simulink model "sf_aircraft"  (R2025b)
settings: configuration reference "SharedConfig" (kept outside this file)
PreLoadFcn:
  | load_system('sf_aircraft_lib.slx');
  | load_system('sf_aircraft_controller.slx');
model workspace (MAT data in the model file):
  reset_cmd = 0
values from neighbouring files (symbols this model uses):
  ActuatorModeType : value not decoded    [sf_aircraft_dd.sldd]
undefined symbols (not defined in the file or in its folder): Left, noise_factor, Right
libraries: simulink x15, sf_aircraft_lib x4, SignalEditorBlockLib x1
(part 2 of 2)

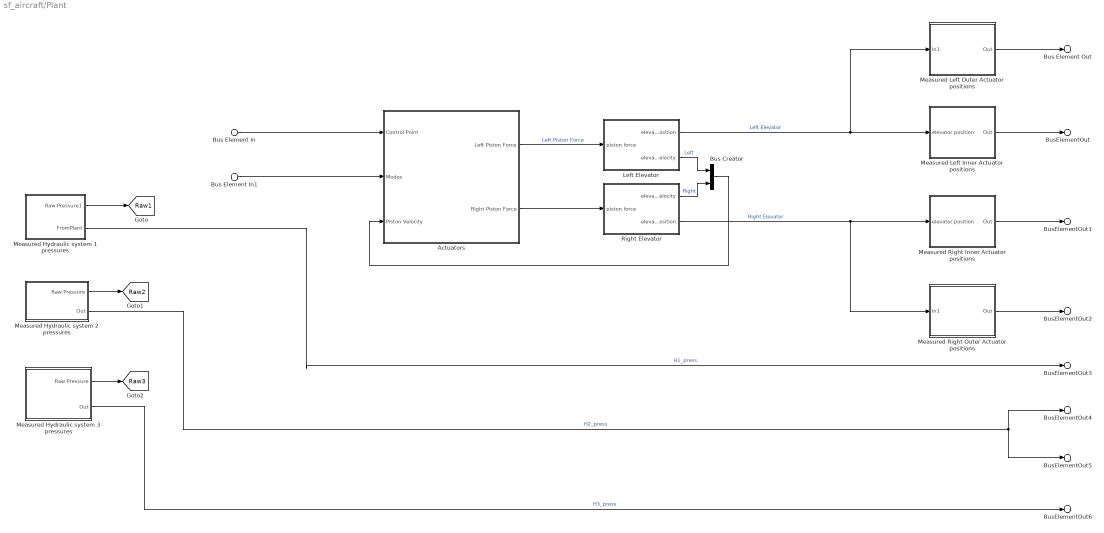
== system sf_aircraft/Plant ==
  Bus Element In : Inport  PortName=To Plant  Element=ControlPoints
  Bus Element In1 : Inport  PortName=To Plant  Element=ActuatorModeCmds
  Actuators : Subsystem
  Bus Creator : BusCreator  Inputs=Left,Right
  Left Elevator : Subsystem
  Measured Hydraulic system 1 pressures : Subsystem
  Measured Hydraulic system 2 pressures : Subsystem
  Measured Hydraulic system 3 pressures : Subsystem
  Measured Left Inner Actuator positions : Subsystem
  Measured Left Outer Actuator positions : Subsystem
  Measured Right Inner Actuator positions : Subsystem
  Measured Right Outer Actuator positions : Subsystem
  Right Elevator : Subsystem
  Bus Element Out : Outport  PortName=FromPlant  Element=PositionReadings.LeftOuterPositionRaw
  BusElementOut : Outport  PortName=FromPlant  Element=PositionReadings.LeftInnerPositionRaw
  BusElementOut1 : Outport  PortName=FromPlant  Element=PositionReadings.RightInnerPositionRaw
  BusElementOut2 : Outport  PortName=FromPlant  Element=PositionReadings.RightOuterPositionRaw
  BusElementOut3 : Outport  PortName=FromPlant  Element=PressureReadings.LeftOuterPressureRaw
  BusElementOut4 : Outport  PortName=FromPlant  Element=PressureReadings.LeftInnerPressureRaw
  BusElementOut5 : Outport  PortName=FromPlant  Element=PressureReadings.RightInnerPressureRaw
  BusElementOut6 : Outport  PortName=FromPlant  Element=PressureReadings.RightOuterPressureRaw
  tag scope: Raw1=global, Raw2=global, Raw3=global
  wires:
  Left Elevator/2(elevator velocity) -> Bus Creator/1  "Left"
  Right Elevator/1(elevator velocity) -> Bus Creator/2  "Right"
  Right Elevator/2(elevator position) -> Measured Right Inner Actuator positions/1(elevator position), Measured Right Outer Actuator positions/1(In1)  "Right Elevator"
  Left Elevator/1(elevator position) -> Measured Left Inner Actuator positions/1(elevator position), Measured Left Outer Actuator positions/1(In1)  "Left Elevator"
  Measured Left Outer Actuator positions/1(Out) -> Bus Element Out/1
  Measured Right Outer Actuator positions/1(Out) -> BusElementOut2/1
  Measured Left Inner Actuator positions/1(Out) -> BusElementOut/1
  Measured Right Inner Actuator positions/1(Out) -> BusElementOut1/1
  Bus Element In/1 -> Actuators/1(Control Point)
  Bus Element In1/1 -> Actuators/2(Modes)
  Measured Hydraulic system 1 pressures/2(FromPlant) -> BusElementOut3/1  "H1_press"
  Measured Hydraulic system 2 pressures/2(Out) -> BusElementOut4/1, BusElementOut5/1  "H2_press"
  Measured Hydraulic system 3 pressures/2(Out) -> BusElementOut6/1  "H3_press"
  Actuators/1(Left Piston Force) -> Left Elevator/1(piston force)  "Left Piston Force"
  Actuators/2(Right Piston Force) -> Right Elevator/1(piston force)
  Bus Creator/1 -> Actuators/3(Piston Velocity)
  Measured Hydraulic system 1 pressures/1(Raw Pressure1) -> [Raw1]
  Measured Hydraulic system 2 pressures/1(Raw Pressure) -> [Raw2]
  Measured Hydraulic system 3 pressures/1(Raw Pressure) -> [Raw3]

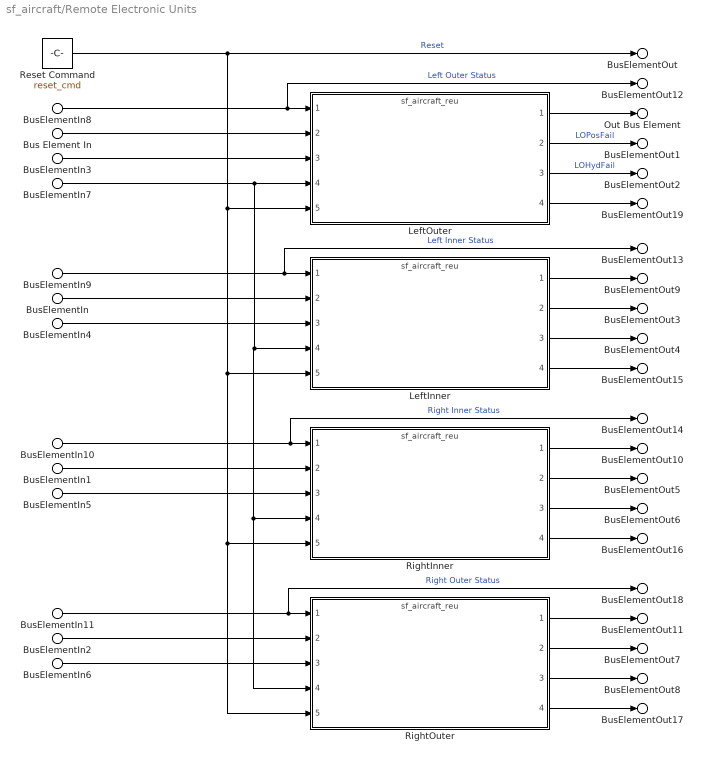
== system sf_aircraft/Remote Electronic Units ==
  BusElementIn7 : Inport  PortName=To REUs  Element=PilotCommand
  BusElementIn8 : Inport  PortName=To REUs  Element=ActuatorModeCmds.LeftOuterMode
  BusElementIn9 : Inport  PortName=To REUs  Element=ActuatorModeCmds.LeftInnerMode
  BusElementIn10 : Inport  PortName=To REUs  Element=ActuatorModeCmds.RightInnerMode
  BusElementIn11 : Inport  PortName=To REUs  Element=ActuatorModeCmds.RightOuterMode
  Bus Element In : Inport  Port=2  PortName=From Plant  Element=PositionReadings.LeftOuterPositionRaw
  BusElementIn : Inport  Port=2  PortName=From Plant  Element=PositionReadings.LeftInnerPositionRaw
  BusElementIn1 : Inport  Port=2  PortName=From Plant  Element=PositionReadings.RightInnerPositionRaw
  BusElementIn2 : Inport  Port=2  PortName=From Plant  Element=PositionReadings.RightOuterPositionRaw
  BusElementIn3 : Inport  Port=2  PortName=From Plant  Element=PressureReadings.LeftOuterPressureRaw
  BusElementIn4 : Inport  Port=2  PortName=From Plant  Element=PressureReadings.LeftInnerPressureRaw
  BusElementIn5 : Inport  Port=2  PortName=From Plant  Element=PressureReadings.RightInnerPressureRaw
  BusElementIn6 : Inport  Port=2  PortName=From Plant  Element=PressureReadings.RightOuterPressureRaw
  LeftInner : ModelReference  ModelNameDialog=sf_aircraft_reu  UsingDefaultArgumentValue=0,0,0,0,0,0,0,0,0,0,0  SimulationMode=Normal  ModelReferenceVersion=1.16
  LeftOuter : ModelReference  ModelNameDialog=sf_aircraft_reu  UsingDefaultArgumentValue=0,0,0,0,0,0,0,0,0,0,0  SimulationMode=Normal  ModelReferenceVersion=1.16
  Reset Command : Constant  Value=reset_cmd  OutDataTypeStr=boolean  SampleTime=.01
  RightInner : ModelReference  ModelNameDialog=sf_aircraft_reu  UsingDefaultArgumentValue=0,0,0,0,0,0,0,0,0,0,0  SimulationMode=Normal  ModelReferenceVersion=1.16
  RightOuter : ModelReference  ModelNameDialog=sf_aircraft_reu  UsingDefaultArgumentValue=0,0,0,0,0,0,0,0,0,0,0  SimulationMode=Normal  ModelReferenceVersion=1.16
  Out Bus Element : Outport  PortName=To Plant  Element=ControlPoints.LeftOuterControlPoint
  BusElementOut9 : Outport  PortName=To Plant  Element=ControlPoints.LeftInnerControlPoint
  BusElementOut10 : Outport  PortName=To Plant  Element=ControlPoints.RightInnerControlPoint
  BusElementOut11 : Outport  PortName=To Plant  Element=ControlPoints.RightOuterControlPoint
  BusElementOut19 : Outport  PortName=To Plant  Element=HydPressures.LeftOuterValidatedHydPressure
  BusElementOut15 : Outport  PortName=To Plant  Element=HydPressures.LeftInnerValidatedPressure
  BusElementOut16 : Outport  PortName=To Plant  Element=HydPressures.RightInnerValidatedPressure
  BusElementOut17 : Outport  PortName=To Plant  Element=HydPressures.RightOuterValidatedPressure
  BusElementOut12 : Outport  PortName=To Plant  Element=ActuatorModeCmds.LeftOuterMode
  BusElementOut13 : Outport  PortName=To Plant  Element=ActuatorModeCmds.LeftInnerMode
  BusElementOut14 : Outport  PortName=To Plant  Element=ActuatorModeCmds.RightInnerMode
  BusElementOut18 : Outport  PortName=To Plant  Element=ActuatorModeCmds.RightOuterMode
  BusElementOut : Outport  Port=2  PortName=From REUs  Element=ResetCmd
  BusElementOut1 : Outport  Port=2  PortName=From REUs  Element=LeftOuterREUout.PositionFailureStatus
  BusElementOut2 : Outport  Port=2  PortName=From REUs  Element=LeftOuterREUout.HydraulicFailureStatus
  BusElementOut3 : Outport  Port=2  PortName=From REUs  Element=LeftInnerREUout.PositionFailureStatus
  BusElementOut4 : Outport  Port=2  PortName=From REUs  Element=LeftInnerREUout.HydraulicFailureStatus
  BusElementOut5 : Outport  Port=2  PortName=From REUs  Element=RightInnerREUout.PositionFailureStatus
  BusElementOut6 : Outport  Port=2  PortName=From REUs  Element=RightInnerREUout.HydraulicFailureStatus
  BusElementOut7 : Outport  Port=2  PortName=From REUs  Element=RightOuterREUout.PositionFailureStatus
  BusElementOut8 : Outport  Port=2  PortName=From REUs  Element=RightOuterREUout.HydraulicFailureStatus
  wires:
  Reset Command/1 -> BusElementOut/1, RightOuter/5, RightInner/5, LeftInner/5, LeftOuter/5  "Reset"
  LeftOuter/2 -> BusElementOut1/1  "LOPosFail"
  LeftOuter/3 -> BusElementOut2/1  "LOHydFail"
  LeftInner/3 -> BusElementOut4/1
  LeftInner/2 -> BusElementOut3/1
  RightInner/2 -> BusElementOut5/1
  RightInner/3 -> BusElementOut6/1
  RightOuter/2 -> BusElementOut7/1
  RightOuter/3 -> BusElementOut8/1
  LeftOuter/1 -> Out Bus Element/1
  LeftInner/1 -> BusElementOut9/1
  RightInner/1 -> BusElementOut10/1
  RightOuter/1 -> BusElementOut11/1
  Bus Element In/1 -> LeftOuter/2
  BusElementIn/1 -> LeftInner/2
  BusElementIn1/1 -> RightInner/2
  BusElementIn2/1 -> RightOuter/2
  BusElementIn3/1 -> LeftOuter/3
  BusElementIn4/1 -> LeftInner/3
  BusElementIn5/1 -> RightInner/3
  BusElementIn6/1 -> RightOuter/3
  BusElementIn7/1 -> LeftOuter/4, RightOuter/4, RightInner/4, LeftInner/4
  BusElementIn8/1 -> BusElementOut12/1, LeftOuter/1  "Left Outer Status"
  BusElementIn9/1 -> BusElementOut13/1, LeftInner/1  "Left Inner Status"
  BusElementIn10/1 -> BusElementOut14/1, RightInner/1  "Right Inner Status"
  BusElementIn11/1 -> BusElementOut18/1, RightOuter/1  "Right Outer Status"
  LeftInner/4 -> BusElementOut15/1
  RightInner/4 -> BusElementOut16/1
  RightOuter/4 -> BusElementOut17/1
  LeftOuter/4 -> BusElementOut19/1

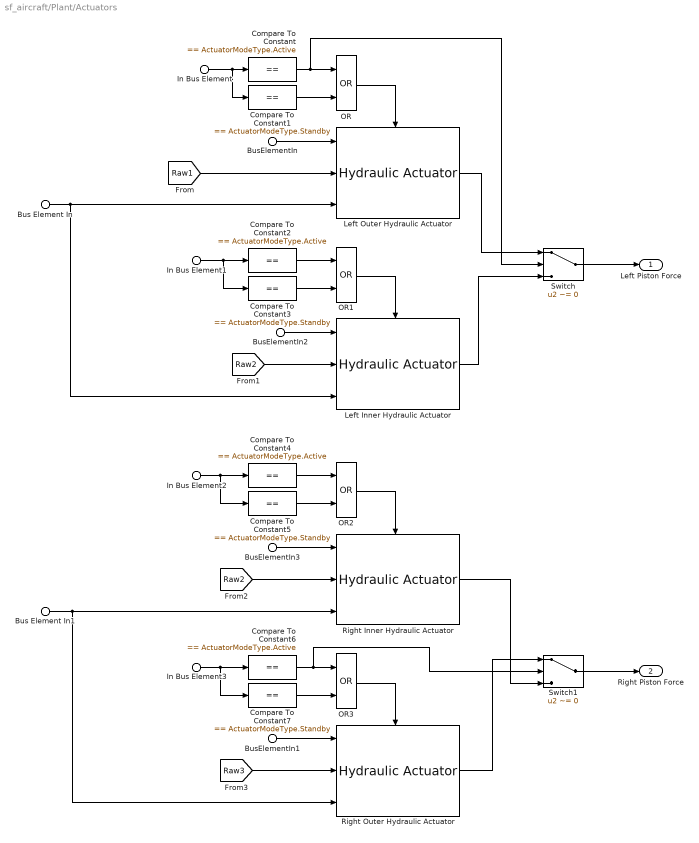
== system sf_aircraft/Plant/Actuators ==
  BusElementIn : Inport  PortName=Control Point  Element=LeftOuterControlPoint
  BusElementIn2 : Inport  PortName=Control Point  Element=LeftInnerControlPoint
  BusElementIn3 : Inport  PortName=Control Point  Element=RightInnerControlPoint
  BusElementIn1 : Inport  PortName=Control Point  Element=RightOuterControlPoint
  In Bus Element : Inport  Port=2  PortName=Modes  Element=LeftOuterMode
  In Bus Element1 : Inport  Port=2  PortName=Modes  Element=LeftInnerMode
  In Bus Element3 : Inport  Port=2  PortName=Modes  Element=RightOuterMode
  In Bus Element2 : Inport  Port=2  PortName=Modes  Element=RightInnerMode
  Bus Element In : Inport  Port=3  PortName=Piston Velocity  Element=Left
  Bus Element In1 : Inport  Port=3  PortName=Piston Velocity  Element=Right
  Compare To Constant{,2,4,6} (4 alike) : simulink/Logic and Bit Operations/Compare To Constant  relop===  const=ActuatorModeType.Active  OutDataTypeStr=boolean
  Compare To Constant{1,3,5,7} (4 alike) : simulink/Logic and Bit Operations/Compare To Constant  relop===  const=ActuatorModeType.Standby  OutDataTypeStr=boolean
  Left Inner Hydraulic Actuator : sf_aircraft_lib/Hydraulic Actuator  SystemSampleTime=-1  VariantActivationTime=update diagram  EmptyChoice=off  PassThrough=off  PassThroughVariantControl=(default)  EmptyChoiceVariantControl=(default)  AllowFlexibleInterface=on  Latency=0  AutoFrameSizeCalculation=off
  Left Outer Hydraulic Actuator : sf_aircraft_lib/Hydraulic Actuator  SystemSampleTime=-1  VariantActivationTime=update diagram  EmptyChoice=off  PassThrough=off  PassThroughVariantControl=(default)  EmptyChoiceVariantControl=(default)  AllowFlexibleInterface=on  Latency=0  AutoFrameSizeCalculation=off
  OR{,1..3} (4 alike) : Logic  Operator=OR  AllPortsSameDT=off  OutDataTypeStr=boolean
  Right Inner Hydraulic Actuator : sf_aircraft_lib/Hydraulic Actuator  SystemSampleTime=-1  VariantActivationTime=update diagram  EmptyChoice=off  PassThrough=off  PassThroughVariantControl=(default)  EmptyChoiceVariantControl=(default)  AllowFlexibleInterface=on  Latency=0  AutoFrameSizeCalculation=off
  Right Outer Hydraulic Actuator : sf_aircraft_lib/Hydraulic Actuator  SystemSampleTime=-1  VariantActivationTime=update diagram  EmptyChoice=off  PassThrough=off  PassThroughVariantControl=(default)  EmptyChoiceVariantControl=(default)  AllowFlexibleInterface=on  Latency=0  AutoFrameSizeCalculation=off
  Switch : Switch  Criteria=u2 ~= 0  SaturateOnIntegerOverflow=off  InputSameDT=off
  Switch1 : Switch  Criteria=u2 ~= 0  SaturateOnIntegerOverflow=off  InputSameDT=off
  Left Piston Force : Outport  VectorParamsAs1DForOutWhenUnconnected=off
  Right Piston Force : Outport  Port=2  VectorParamsAs1DForOutWhenUnconnected=off
  wires:
  BusElementIn/1 -> Left Outer Hydraulic Actuator/1
  [Raw1] -> Left Outer Hydraulic Actuator/2
  In Bus Element/1 -> Compare To Constant1/1, Compare To Constant/1
  Compare To Constant/1 -> Switch/2, OR/1
  Compare To Constant1/1 -> OR/2
  OR/1 -> Left Outer Hydraulic Actuator/Enable
  OR1/1 -> Left Inner Hydraulic Actuator/Enable
  Compare To Constant2/1 -> OR1/1
  Compare To Constant3/1 -> OR1/2
  In Bus Element1/1 -> Compare To Constant3/1, Compare To Constant2/1
  [Raw2] -> Left Inner Hydraulic Actuator/2
  BusElementIn2/1 -> Left Inner Hydraulic Actuator/1
  Bus Element In/1 -> Left Inner Hydraulic Actuator/3, Left Outer Hydraulic Actuator/3
  Compare To Constant6/1 -> Switch1/2, OR3/1
  Compare To Constant7/1 -> OR3/2
  OR3/1 -> Right Outer Hydraulic Actuator/Enable
  OR2/1 -> Right Inner Hydraulic Actuator/Enable
  Compare To Constant4/1 -> OR2/1
  Compare To Constant5/1 -> OR2/2
  BusElementIn3/1 -> Right Inner Hydraulic Actuator/1
  In Bus Element2/1 -> Compare To Constant5/1, Compare To Constant4/1
  In Bus Element3/1 -> Compare To Constant7/1, Compare To Constant6/1
  [Raw3] -> Right Outer Hydraulic Actuator/2
  BusElementIn1/1 -> Right Outer Hydraulic Actuator/1
  Bus Element In1/1 -> Right Outer Hydraulic Actuator/3, Right Inner Hydraulic Actuator/3
  Left Outer Hydraulic Actuator/1 -> Switch/1
  Left Inner Hydraulic Actuator/1 -> Switch/3
  Switch/1 -> Left Piston Force/1
  Switch1/1 -> Right Piston Force/1
  Right Inner Hydraulic Actuator/1 -> Switch1/3
  Right Outer Hydraulic Actuator/1 -> Switch1/1
  [Raw2] -> Right Inner Hydraulic Actuator/2

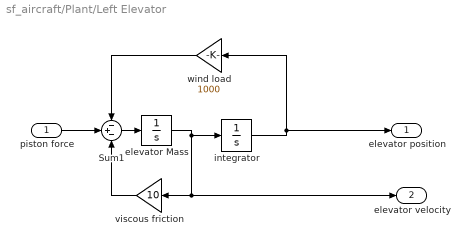
== system sf_aircraft/Plant/Left Elevator ==
  piston force : Inport
  Sum1 : Sum  Inputs=-+-  SaturateOnIntegerOverflow=on
  elevator Mass : Integrator  LimitOutput=on  UpperSaturationLimit=5  LowerSaturationLimit=-5
  integrator : Integrator  LimitOutput=on  UpperSaturationLimit=2  LowerSaturationLimit=-2
  viscous friction : Gain  Gain=10  SaturateOnIntegerOverflow=on  OutDataTypeStr=Inherit: Same as input  ParamDataTypeStr=Inherit: Same as input
  wind load : Gain  Gain=1000  SaturateOnIntegerOverflow=on  OutDataTypeStr=Inherit: Same as input  ParamDataTypeStr=Inherit: Same as input
  elevator position : Outport  VectorParamsAs1DForOutWhenUnconnected=off
  elevator velocity : Outport  Port=2  VectorParamsAs1DForOutWhenUnconnected=off
  wires:
  Sum1/1 -> elevator Mass/1
  elevator Mass/1 -> viscous friction/1, elevator velocity/1, integrator/1
  integrator/1 -> wind load/1, elevator position/1
  piston force/1 -> Sum1/2
  viscous friction/1 -> Sum1/3
  wind load/1 -> Sum1/1

== system sf_aircraft/Plant/Measured Hydraulic system 1 pressures ==
  Hydraulic pressure1 : Subsystem
  pressure reading1 : Subsystem
  Raw Pressure1 : Outport
  FromPlant : Outport  Port=2  VectorParamsAs1DForOutWhenUnconnected=off
  wires:
  Hydraulic pressure1/1(Raw Pressure) -> Raw Pressure1/1, pressure reading1/1(pressure)
  pressure reading1/1(Out) -> FromPlant/1

== system sf_aircraft/Plant/Measured Hydraulic system 2 pressures ==
  Hydraulic pressure : Subsystem
  pressure reading2 : Subsystem
  Raw Pressure : Outport
  Out : Outport  Port=2  VectorParamsAs1DForOutWhenUnconnected=off
  wires:
  Hydraulic pressure/1(Raw Pressure) -> Raw Pressure/1, pressure reading2/1(pressure)
  pressure reading2/1(Out) -> Out/1

== system sf_aircraft/Plant/Measured Hydraulic system 3 pressures ==
  Hydraulic pressure : Subsystem
  pressure reading3 : Subsystem
  Raw Pressure : Outport
  Out : Outport  Port=2  VectorParamsAs1DForOutWhenUnconnected=off
  wires:
  Hydraulic pressure/1(Raw Pressure) -> Raw Pressure/1, pressure reading3/1(pressure)
  pressure reading3/1(Out) -> Out/1

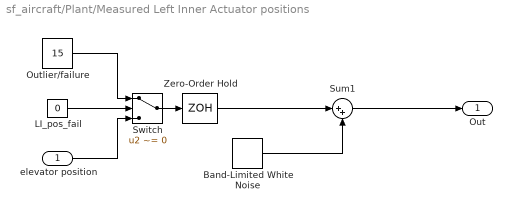
== system sf_aircraft/Plant/Measured Left Inner Actuator positions ==
  elevator position : Inport
  Band-Limited White Noise : simulink/Sources/Band-Limited White Noise  Cov=[0.00001 0.00001 0.00001]*noise_factor  Ts=.1  seed=[23651]
  LI_pos_fail : Constant  Value=0  OutDataTypeStr=boolean  SampleTime=.01
  Outlier/failure : Constant  Value=15  SampleTime=.01
  Sum1 : Sum  Inputs=|++  SaturateOnIntegerOverflow=on
  Switch : Switch  Criteria=u2 ~= 0  InputSameDT=off
  Zero-Order Hold : ZeroOrderHold  SampleTime=-1
  Out : Outport  VectorParamsAs1DForOutWhenUnconnected=off
  wires:
  Switch/1 -> Zero-Order Hold/1
  Outlier/failure/1 -> Switch/1
  LI_pos_fail/1 -> Switch/2
  elevator position/1 -> Switch/3
  Sum1/1 -> Out/1
  Zero-Order Hold/1 -> Sum1/1
  Band-Limited White Noise/1 -> Sum1/2

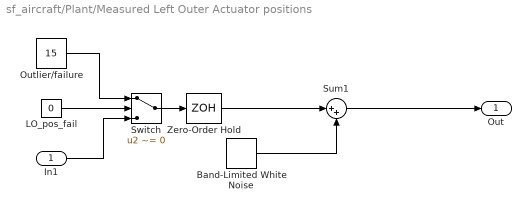
== system sf_aircraft/Plant/Measured Left Outer Actuator positions ==
  In1 : Inport
  Band-Limited White Noise : simulink/Sources/Band-Limited White Noise  Cov=[0.00001 0.00001 0.00001]*noise_factor  Ts=0.1  seed=[23341]
  LO_pos_fail : Constant  Value=0  OutDataTypeStr=boolean  SampleTime=.01
  Outlier/failure : Constant  Value=15  SampleTime=.01
  Sum1 : Sum  Inputs=|++  SaturateOnIntegerOverflow=on
  Switch : Switch  Criteria=u2 ~= 0  InputSameDT=off
  Zero-Order Hold : ZeroOrderHold  SampleTime=-1
  Out : Outport  VectorParamsAs1DForOutWhenUnconnected=off
  wires:
  Sum1/1 -> Out/1
  Switch/1 -> Zero-Order Hold/1
  Outlier/failure/1 -> Switch/1
  LO_pos_fail/1 -> Switch/2
  In1/1 -> Switch/3
  Band-Limited White Noise/1 -> Sum1/2
  Zero-Order Hold/1 -> Sum1/1

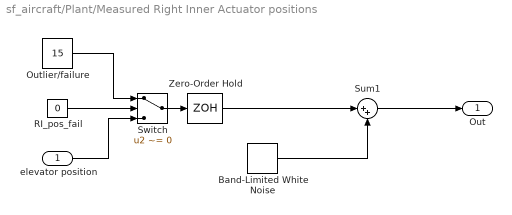
== system sf_aircraft/Plant/Measured Right Inner Actuator positions ==
  elevator position : Inport
  Band-Limited White Noise : simulink/Sources/Band-Limited White Noise  Cov=[0.00001 0.00001 0.00001]*noise_factor  Ts=.1  seed=[13651]
  Outlier/failure : Constant  Value=15  SampleTime=.01
  RI_pos_fail : Constant  Value=0  OutDataTypeStr=boolean  SampleTime=.01
  Sum1 : Sum  Inputs=|++  SaturateOnIntegerOverflow=on
  Switch : Switch  Criteria=u2 ~= 0  InputSameDT=off
  Zero-Order Hold : ZeroOrderHold  SampleTime=-1
  Out : Outport  VectorParamsAs1DForOutWhenUnconnected=off
  wires:
  Switch/1 -> Zero-Order Hold/1
  Sum1/1 -> Out/1
  Outlier/failure/1 -> Switch/1
  RI_pos_fail/1 -> Switch/2
  elevator position/1 -> Switch/3
  Band-Limited White Noise/1 -> Sum1/2
  Zero-Order Hold/1 -> Sum1/1

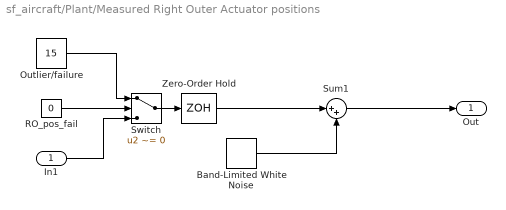
== system sf_aircraft/Plant/Measured Right Outer Actuator positions ==
  In1 : Inport
  Band-Limited White Noise : simulink/Sources/Band-Limited White Noise  Cov=[0.00001 0.00001 0.00001]*noise_factor  Ts=.1  seed=[13651]
  Outlier/failure : Constant  Value=15  SampleTime=.01
  RO_pos_fail : Constant  Value=0  OutDataTypeStr=boolean  SampleTime=.01
  Sum1 : Sum  Inputs=|++  SaturateOnIntegerOverflow=on
  Switch : Switch  Criteria=u2 ~= 0  InputSameDT=off
  Zero-Order Hold : ZeroOrderHold  SampleTime=-1
  Out : Outport  VectorParamsAs1DForOutWhenUnconnected=off
  wires:
  In1/1 -> Switch/3
  RO_pos_fail/1 -> Switch/2
  Outlier/failure/1 -> Switch/1
  Switch/1 -> Zero-Order Hold/1
  Zero-Order Hold/1 -> Sum1/1
  Sum1/1 -> Out/1
  Band-Limited White Noise/1 -> Sum1/2

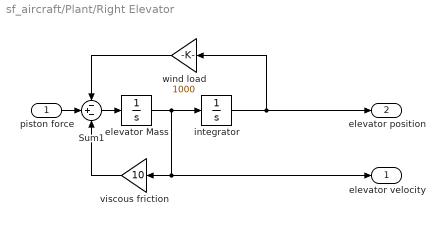
== system sf_aircraft/Plant/Right Elevator ==
  piston force : Inport
  Sum1 : Sum  Inputs=-+-  SaturateOnIntegerOverflow=on
  elevator Mass : Integrator
  integrator : Integrator
  viscous friction : Gain  Gain=10  SaturateOnIntegerOverflow=on  OutDataTypeStr=Inherit: Same as input  ParamDataTypeStr=Inherit: Same as input
  wind load : Gain  Gain=1000  SaturateOnIntegerOverflow=on  OutDataTypeStr=Inherit: Same as input  ParamDataTypeStr=Inherit: Same as input
  elevator velocity : Outport  VectorParamsAs1DForOutWhenUnconnected=off
  elevator position : Outport  Port=2  VectorParamsAs1DForOutWhenUnconnected=off
  wires:
  integrator/1 -> elevator position/1, wind load/1
  elevator Mass/1 -> integrator/1, viscous friction/1, elevator velocity/1
  Sum1/1 -> elevator Mass/1
  wind load/1 -> Sum1/1
  viscous friction/1 -> Sum1/3
  piston force/1 -> Sum1/2

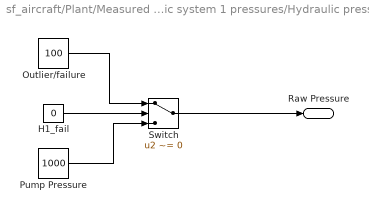
== system sf_aircraft/Plant/Measured Hydraulic system 1 pressures/Hydraulic pressure1 ==
  H1_fail : Constant  Value=0  OutDataTypeStr=boolean  SampleTime=.01
  Outlier/failure : Constant  Value=100  SampleTime=.01
  Pump Pressure : Constant  Value=1000  SampleTime=.01
  Switch : Switch  Criteria=u2 ~= 0  InputSameDT=off
  Raw Pressure : Outport  VectorParamsAs1DForOutWhenUnconnected=off
  wires:
  Pump Pressure/1 -> Switch/3
  Switch/1 -> Raw Pressure/1
  Outlier/failure/1 -> Switch/1
  H1_fail/1 -> Switch/2

== system sf_aircraft/Plant/Measured Hydraulic system 1 pressures/pressure reading1 ==
  pressure : Inport
  Band-Limited White Noise : simulink/Sources/Band-Limited White Noise  Cov="[0.1 0.1  0.1]*noise_factor"  Ts=.01  seed=[25341]
  Sum : Sum  Inputs=|++  SaturateOnIntegerOverflow=on
  Out : Outport  VectorParamsAs1DForOutWhenUnconnected=off
  wires:
  Band-Limited White Noise/1 -> Sum/2
  pressure/1 -> Sum/1
  Sum/1 -> Out/1

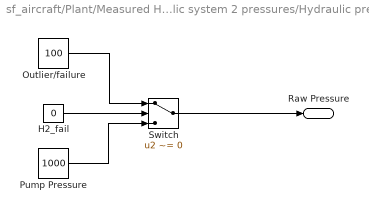
== system sf_aircraft/Plant/Measured Hydraulic system 2 pressures/Hydraulic pressure ==
  H2_fail : Constant  Value=0  OutDataTypeStr=boolean  SampleTime=.01
  Outlier/failure : Constant  Value=100  SampleTime=.01
  Pump Pressure : Constant  Value=1000  SampleTime=.01
  Switch : Switch  Criteria=u2 ~= 0  InputSameDT=off
  Raw Pressure : Outport  VectorParamsAs1DForOutWhenUnconnected=off
  wires:
  Pump Pressure/1 -> Switch/3
  Switch/1 -> Raw Pressure/1
  Outlier/failure/1 -> Switch/1
  H2_fail/1 -> Switch/2

== system sf_aircraft/Plant/Measured Hydraulic system 2 pressures/pressure reading2 ==
  pressure : Inport
  Band-Limited White Noise : simulink/Sources/Band-Limited White Noise  Cov="[0.1 0.1  0.1]*noise_factor"  Ts=.01  seed=[25341]
  Sum : Sum  Inputs=|++  SaturateOnIntegerOverflow=on
  Out : Outport  VectorParamsAs1DForOutWhenUnconnected=off
  wires:
  Band-Limited White Noise/1 -> Sum/2
  pressure/1 -> Sum/1
  Sum/1 -> Out/1

== system sf_aircraft/Plant/Measured Hydraulic system 3 pressures/Hydraulic pressure ==
  H3_fail : Constant  Value=0  OutDataTypeStr=boolean  SampleTime=.01
  Outlier/failure : Constant  Value=100  SampleTime=.01
  Pump Pressure : Constant  Value=1000  SampleTime=.01
  Switch : Switch  Criteria=u2 ~= 0  InputSameDT=off
  Raw Pressure : Outport  VectorParamsAs1DForOutWhenUnconnected=off
  wires:
  Pump Pressure/1 -> Switch/3
  Switch/1 -> Raw Pressure/1
  Outlier/failure/1 -> Switch/1
  H3_fail/1 -> Switch/2

== system sf_aircraft/Plant/Measured Hydraulic system 3 pressures/pressure reading3 ==
  pressure : Inport
  Band-Limited White Noise : simulink/Sources/Band-Limited White Noise  Cov="[0.1 0.1  0.1]*noise_factor"  Ts=.01  seed=[25341]
  Sum : Sum  Inputs=|++  SaturateOnIntegerOverflow=on
  Out : Outport  VectorParamsAs1DForOutWhenUnconnected=off
  wires:
  Band-Limited White Noise/1 -> Sum/2
  pressure/1 -> Sum/1
  Sum/1 -> Out/1
